simulink model "orig_exp_second_order"  (R2023a)
settings: Solver=ode4  StartTime=0.0  StopTime=20  FixedStep=0.0005  RelTol=1e-3
settings Model: Creator=Anonymous  LastModifiedBy=Anonymous

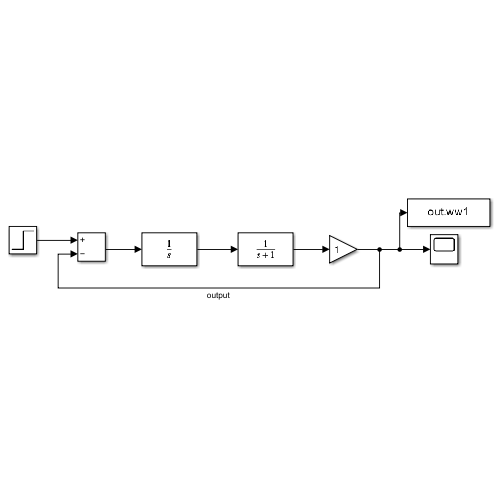
[thumbnail: Simulink's stored preview of the top-level diagram]
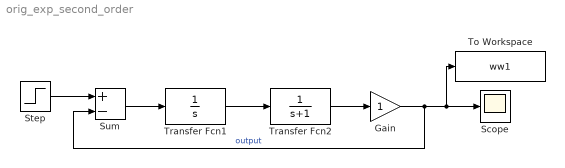
== system orig_exp_second_order ==
  Gain : Gain
  Scope : Scope
  Step : Step  SampleTime=0
  Sum : Sum  Inputs=+-
  To Workspace : ToWorkspace  VariableName=ww1  SaveFormat=Timeseries  SampleTime=-1
  Transfer Fcn1 : TransferFcn  Numerator=1  Denominator=[1 0]
  Transfer Fcn2 : TransferFcn  Numerator=1  Denominator=[1 1]
  wires:
  Gain/1 -> Sum/2, To Workspace/1, Scope/1  "output"
  Transfer Fcn2/1 -> Gain/1
  Transfer Fcn1/1 -> Transfer Fcn2/1
  Sum/1 -> Transfer Fcn1/1
  Step/1 -> Sum/1
